simulink model "mimo_4x4_zf"  (R2024b)
settings: Solver=FixedStepDiscrete  StartTime=0  StopTime=0  FixedStep=1  RelTol=1e-3
settings Model: Creator=Devansh  LastModifiedBy=Devansh
settings DataIOCC: SaveOutput=off  SignalLogging=off  SaveTime=off  ReturnWorkspaceOutputs=off

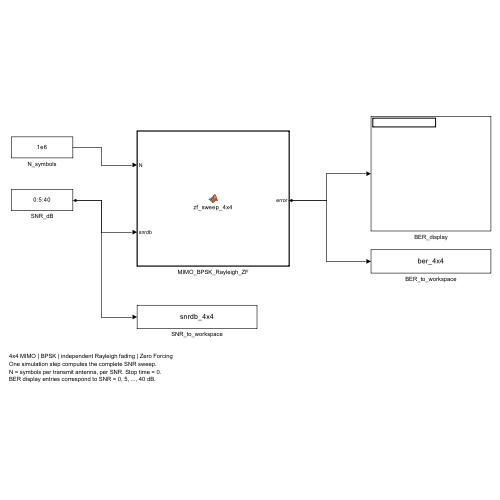
[thumbnail: Simulink's stored preview of the top-level diagram]
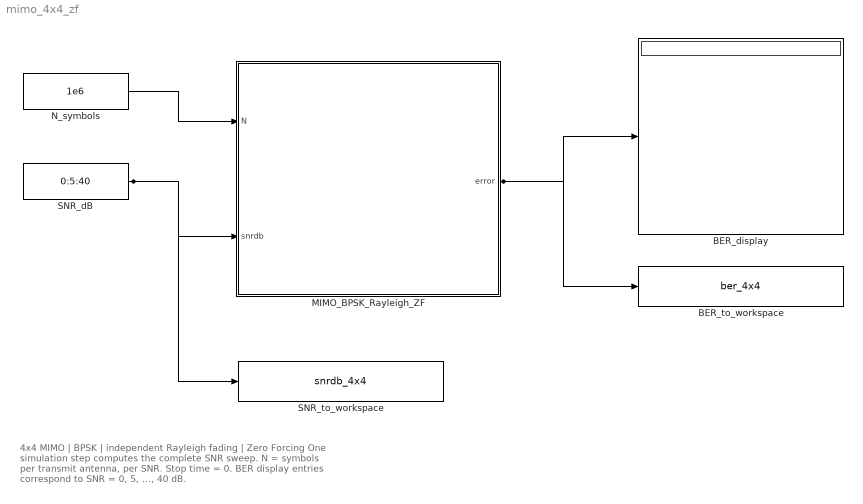
== system mimo_4x4_zf ==
  note: 4x4 MIMO | BPSK | independent Rayleigh fading | Zero Forcing
      | One simulation step computes the complete SNR sweep.
      | N = symbols per transmit antenna, per SNR. Stop time = 0.
      | BER display entries correspond to SNR = 0, 5, ..., 40 dB.
  BER_display : Display
  BER_to_workspace : ToWorkspace  VariableName=ber_4x4  SampleTime=-1
  MIMO_BPSK_Rayleigh_ZF : MATLAB Function  TreatAsAtomicUnit=on
  N_symbols : Constant  Value=1e6  SampleTime=1
  SNR_dB : Constant  Value=0:5:40  SampleTime=1
  SNR_to_workspace : ToWorkspace  VariableName=snrdb_4x4  SampleTime=-1
  wires:
  N_symbols/1 -> MIMO_BPSK_Rayleigh_ZF/1(N)
  SNR_dB/1 -> MIMO_BPSK_Rayleigh_ZF/2(snrdb), SNR_to_workspace/1
  MIMO_BPSK_Rayleigh_ZF/1(error) -> BER_display/1, BER_to_workspace/1

== matlab function mimo_4x4_zf/MIMO_BPSK_Rayleigh_ZF ==
  data: N input; error output; snrdb input
function error = zf_sweep_4x4(N, snrdb)
%#codegen
% Original script calculation; N and snrdb are Constant block inputs.
Nt = 4;
Nr = 4;
snrlinear = 10.^(snrdb/10);
nsd = 1 ./ sqrt(snrlinear);
error = zeros(size(snrdb));
for j = 1:length(snrdb)
    x11 = randi([0 1],Nt,N);
    X = 2*x11-1;
    H = (randn(Nr,Nt,N)+1j*randn(Nr,Nt,N))/sqrt(2);
    noise = (randn(Nr,N)+1j*randn(Nr,N))/sqrt(2);
    % Explicit complex allocation for MATLAB Function code generation.
    Y = complex(zeros(Nr,N));
    xest = complex(zeros(Nt,N));
    for i = 1:N
        Y(:,i) = H(:,:,i)*X(:,i)+noise(:,i)*nsd(j);
        xest(:,i) = H(:,:,i)\Y(:,i);
    end
    x_detected = 2*(real(xest)>0)-1;
    error(j) = sum(X(:)~=x_detected(:))/(Nt*N);
end
end
